simulink model "MC710_ID2"  (Simulink 7.2)
settings: Solver=FixedStepDiscrete  StartTime=0.0  StopTime=5  FixedStep=0.002  RelTol=1e-3
undefined symbols (not defined in the file or in its folder): OC2max, QEIInit, sendPOS, y1
libraries: dsPICdrivers x10, simulink x1
settings Model: Creator=ASL_Lab  LastModifiedBy=magicNTU
settings OptimizationCC: InlineParams=on  InlineInvariantSignals=on  InitFltsAndDblsToZero=on  OptimizeModelRefInitCode=on  LifeSpan=1
settings DebuggingCC: SaveWithParameterizedLinksMsg=none
settings HardwareCC: ProdBitPerInt=16  ProdEndianess=LittleEndian  ProdWordSize=16  ProdHWDeviceType=16-bit Generic
settings RTWCC: SystemTargetFile=dspic.tlc  TemplateMakefile=dspic_pic30_gcc.tmf  PostCodeGenCommand=dsPIC_Compile()  Description=Embedded Target for Microchip dsPIC (real-time)  GenerateReport=on  ProcessScript=dspic_make_rtw_hook  CustomSource=QEI_ID.c  IncludeHyperlinkInReport=on  LaunchReport=on  GenerateTraceInfo=on  GenerateTraceReport=on  GenerateTraceReportSl=on  GenerateTraceReportSf=on  GenerateTraceReportEml=on
settings CodeAppCC: IgnoreCustomStorageClasses=off
settings STFCustomTargetCC: ModelReferenceCompliant=off  IncludeMdlTerminateFcn=off  CombineOutputUpdateFcns=on  SuppressErrorStatus=on  ERTCustomFileBanners=on  SupportContinuousTime=off  SupportNonInlinedSFcns=off  SystemTargetFile=dspic.tlc
settings ERTTargetCC: MultiwordLength=2048  ModelReferenceCompliant=off  CompOptLevelCompliant=off  IncludeMdlTerminateFcn=off  SuppressErrorStatus=on  ERTFirstTimeCompliant=off  ModelStepFunctionPrototypeControlCompliant=off  CPPClassGenCompliant=off  ExtModeMexFile=noextcomm  InlinedParameterPlacement=NonHierarchical  ERTSrcFileBannerTemplate=dsPIC_code_template.cgt  ERTHdrFileBannerTemplate=dsPIC_code_template.cgt  ERTDataSrcFileTemplate=dsPIC_code_template.cgt  ERTDataHdrFileTemplate=dsPIC_code_template.cgt  ERTCustomFileTemplate=dsPIC_main.tlc
settings CustomProperty: DataType=string  Value=C:\PROGRA~1\MATLAB\R2008b\bin\win32\gmake

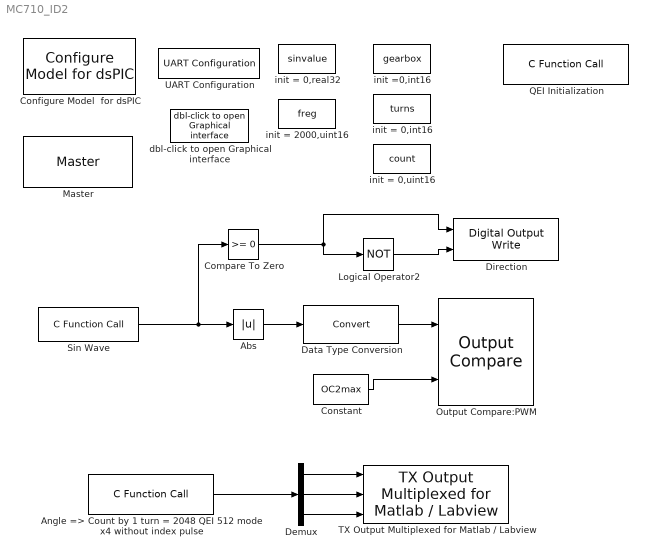
== system MC710_ID2 ==
  Abs : Abs  OutDataType=sfix(16)  OutScaling=2^0
  Angle => Count by 1 turn = 2048 QEI 512 mode x4 without index pulse : dsPICdrivers/OTHERS/C Function Call  Tag=dsPIC_dsPIC_CFunctionCall  fctName='sendPOS'  INPUT_SIZE=1  INPUT1=--  INPUT2=--  INPUT3=--  OUTPUT_SIZE=3  OUTPUT1=int16  SampleTime=.002  InputType=[ ]  OutputType=[ 3 ]  FctDeclaration=extern void sendPOS(int16_T* y1);  FctCall=sendPOS(*%y1);  OrderingInOutPopup=None
  Compare To Zero : simulink/Logic and Bit Operations/Compare To Zero  SystemSampleTime=-1  relop=>=  LogicOutDataTypeMode=boolean  ZeroCross=off
  Configure Model  for dsPIC : dsPICdrivers/Simulink Configuration/Configure Model  for dsPIC
  Constant : Constant  Value=OC2max  OutDataTypeMode=uint16  OutDataType=sfix(16)  OutScaling=2^0  OutDataTypeStr=uint16
  Data Type Conversion : DataTypeConversion  OutDataType=sfix(16)  OutScaling=2^0
  Demux : Demux  Outputs=3
  Direction : dsPICdrivers/Digital I//O/Digital Output Write  Tag=dsPIC_Digital_Output  Priority=5  PORT=F  Pin=[2 3]  Simultaneous=off  OrderingInOutPopup=None
  Logical Operator2 : Logic  Operator=NOT  Inputs=1  OutDataTypeMode=boolean  OutDataTypeStr=boolean
  Master : dsPICdrivers/Master  Tag=dsPIC_MASTER  TimeStepType=Timer1  picType=33fJ256MC710  fcy=27600000  Quartz_33f=20e6  PLLActive_33f=on  fcyDesired_33f=27600000  tmr1="[1  55199  0]"  tmr1Info="Time Step : 0.002  ;   Error : 0%  PR1=55199"  tmr2345="[1  0  0  0  0  0  0  0]"  tmr2345cfg=[-1 -1 -1 -1 -1 -1 -1 -1]  IOautoConf=on  typePort="[ 0   0   0   0   0   0   0   0   0   0   0   0   0   0   0   0   0   0   0   0   0   0   0   0   0   0   0   0   0   0   0   0   0   0   0   0   0   0   0   0   0   0   0   0   0   0   0   0   0   7   0   0   0   0   0   0   0   0   0   0   0   0   0   0   0   0   0   0   0   0   0   0   0   0   0   0   0   0   0   0   0   0  10  10   4   5   0   0   0   0   0   0   0   0   0   0   0   0   0   0   0   0   0   0   0   0   0   0   0   0   0   0 ]"  TRIS="[ 65535  65535  65535  65533  65535  65523  65535 ]"  ADPCFG=0  MasterBusyPort=None  MasterOverloadPort=None  FOSC=Quartz (XT - HS)  ClockSwitchMonitor=Both disabled  TempProtection_33f=TEMP_ON  FPBOR=<empty>  PWRT=64ms  MCLR=<empty>  PowerSave=off  OverrideFcy=off  NewFcy=1e6
  Output Compare:PWM : dsPICdrivers/Peripheral I//O/Output Compare  Tag=dsPIC_PWM_out  Priority=5  IntPriority=3  CHANNEL=[2]  Channel_UP_Down_Periode=[5]  MaxChannel=[5e-005]  MaxName=' OC2max '  Precision=[10.4305]  Timer=[2]  Status=OK  SafeMarge=[0]  PortLetter=[68]  PortNumber=[1]  MaxValues=[1380]
  QEI Initialization : dsPICdrivers/OTHERS/C Function Call  Tag=dsPIC_dsPIC_CFunctionCall  fctName='QEIInit'  INPUT_SIZE=1  INPUT1=--  INPUT2=--  INPUT3=--  OUTPUT_SIZE=1  OUTPUT1=--  SampleTime=inf  InputType=[ ]  OutputType=[ ]  FctDeclaration=extern void QEIInit();  FctCall=QEIInit();  OrderingInOutPopup=None
  Sin Wave : dsPICdrivers/OTHERS/C Function Call  Tag=dsPIC_dsPIC_CFunctionCall  fctName='sinout'  INPUT_SIZE=1  INPUT1=--  INPUT2=--  INPUT3=--  OUTPUT_SIZE=1  OUTPUT1=real32  SampleTime=.002  InputType=[ ]  OutputType=[ 7 ]  FctDeclaration=extern real32_T sinout();  FctCall=%y1 = sinout();  OrderingInOutPopup=None
  TX Output Multiplexed for Matlab / Labview : dsPICdrivers/Serial PORT/TX Output Multiplexed for Matlab // Labview  Tag=dsPIC_TX_Multiplexed  Priority=5  UART=2  CleverSpreadingChk=on  CleverSpreading=1  CHANNEL=[0 1 2]  CHANNELBLOCKED=[]  CHANNELBLOCKED_BITEWISE=0  Status=OK
  UART Configuration : dsPICdrivers/Serial PORT/UART Configuration  Tag=dsPIC_config_UART  UART=2  proposed_BAUD=115200  ALT_TX_RX=off  InterruptTxWhen=When Transmit Buffer is empty  TXInterruptPri=7  TxBufferSize=32  TXEN=on  InterruptRxWhen=When Receive Buffer is full (contain 4 characters)  RXInterruptPri=1  RxBufferSize=4  BAUD=115200  UxBRG=14  Info="UxBRG = 14   ||  Real Baud : 115000   ||  % error : -0.17361  ||  max 23 Bytes / Step"  RealBaud=0
  dbl-click to open Graphical interface : dsPICdrivers/Serial PORT/dbl-click to open Graphical interface  SystemSampleTime=-1  Nothing=0
  init = 0,int16 : DataStoreMemory  DataStoreName=turns  ReadBeforeWriteMsg=warning  WriteAfterWriteMsg=warning  WriteAfterReadMsg=warning  DataType=int16  OutDataType=sfix(16)  OutScaling=2^0  OutDataTypeStr=int16
      settings: RTWStateStorageClass=ExportedGlobal
  init = 0,real32 : DataStoreMemory  DataStoreName=sinvalue  ReadBeforeWriteMsg=warning  WriteAfterWriteMsg=warning  WriteAfterReadMsg=warning  DataType=single  OutDataType=sfix(16)  OutScaling=2^0  OutDataTypeStr=single
      settings: RTWStateStorageClass=ExportedGlobal
  init = 0,uint16 : DataStoreMemory  DataStoreName=count  ReadBeforeWriteMsg=warning  WriteAfterWriteMsg=warning  WriteAfterReadMsg=warning  DataType=uint16  OutDataType=sfix(16)  OutScaling=2^0  OutDataTypeStr=uint16
      settings: RTWStateStorageClass=ExportedGlobal
  init = 2000,uint16 : DataStoreMemory  DataStoreName=freg  ReadBeforeWriteMsg=warning  WriteAfterWriteMsg=warning  WriteAfterReadMsg=warning  InitialValue=2000  DataType=uint16  OutDataType=sfix(16)  OutScaling=2^0  OutDataTypeStr=uint16
      settings: RTWStateStorageClass=ExportedGlobal
  init =0,int16 : DataStoreMemory  DataStoreName=gearbox  ReadBeforeWriteMsg=warning  WriteAfterWriteMsg=warning  WriteAfterReadMsg=warning  DataType=int16  OutDataType=sfix(16)  OutScaling=2^0  OutDataTypeStr=int16
      settings: RTWStateStorageClass=ExportedGlobal
  wires:
  Constant/1 -> Output Compare:PWM/2
  Data Type Conversion/1 -> Output Compare:PWM/1
  Sin Wave/1 -> Abs/1, Compare To Zero/1
  Compare To Zero/1 -> Logical Operator2/1, Direction/1
  Abs/1 -> Data Type Conversion/1
  Logical Operator2/1 -> Direction/2
  Demux/1 -> TX Output Multiplexed for Matlab / Labview/1
  Angle => Count by 1 turn = 2048 QEI 512 mode x4 without index pulse/1 -> Demux/1
  Demux/2 -> TX Output Multiplexed for Matlab / Labview/2
  Demux/3 -> TX Output Multiplexed for Matlab / Labview/3
